simulink model "Homodyne_Tranceriver_model_v2"  (R2026b)
settings: Solver=VariableStepAuto  StopTime=16
libraries: fl_lib x10, nesl_utility x5, simrfV2util1 x4, simrfV2elements x4, simrfV2_lib x2, ee_lib x2, dspsigops x1, simulink_extras x1, simulink x1
settings Model: Creator=dylan  LastModifiedBy=dylan
settings SimscapeCC: SimscapeLogType=all  SimscapeNominalValues="[{\"value\":\"1\",\"unit\":\"A\"},{\"value\":\"1\",\"unit\":\"bar\"},{\"value\":\"1\",\"unit\":\"cm^2\"},{\"value\":\"1\",\"unit\":\"cm^3/s\"},{\"value\":\"1\",\"unit\":\"kJ/kg\"},{\"value\":\"1\",\"unit\":\"kW\"},{\"value\":\"1\",\"unit\":\"l\"},{\"value\":\"1\",\"unit\":\"N\"},{\"value\":\"1\",\"unit\":\"N*m\"},{\"value\":\"1\",\"unit\":\"V\"},{\"value\":\"0.001\",\"unit\":\"Wb\"}]"  SimscapeUseEnergyAccounting=off

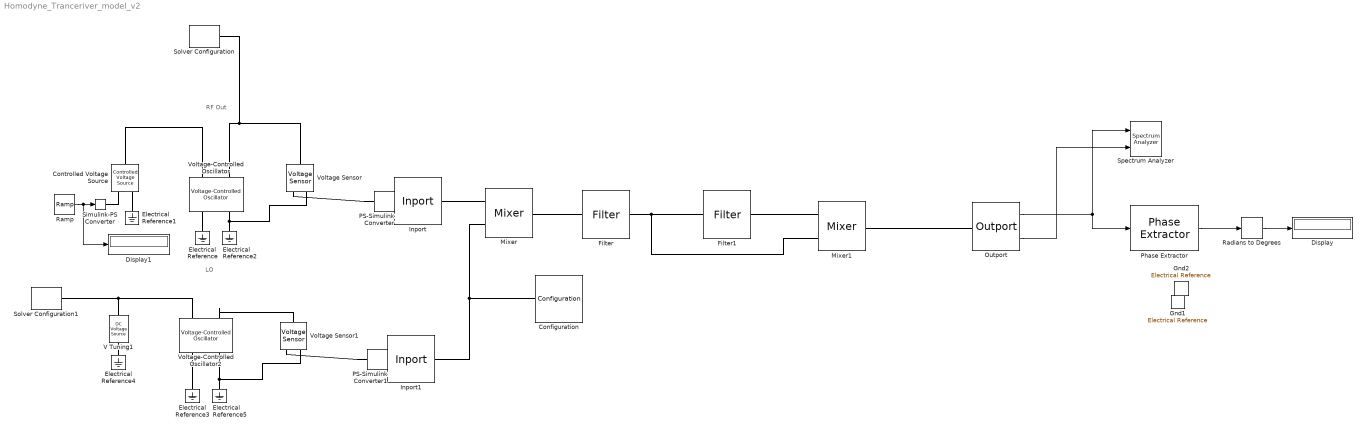
== system Homodyne_Tranceriver_model_v2 ==
  note: RF Out
  note: LO
  Configuration : simrfV2util1/Configuration  AutoFreq=on  Tones=[0] Hz  Harmonics=[1]  NormalizeCarrierPower=on  SolverType=Auto  UseCCode=on  StepSize=1 ns  AddNoise=on  defaultRNG=on  Seed=0  Temperature=290.0 K  SolverDelFlag=0  AbsTol=1e-6  RelTol=1e-3  MaxIter=10  ErrorEstimationType=2-norm over all variables  EnableInterpFilter=on  HiddenFIRfilterControllerParam=off  SmallSignalApprox=off  AllSimFreqs=on  SimFreqs=[] Hz  SimFreqsInternal=[]  SamplesPerFrame=1
  Controlled Voltage Source : fl_lib/Electrical/Electrical Sources/Controlled Voltage Source
  Display : Display
  Display1 : Display
  Electrical Reference{,1..5} (6 alike) : fl_lib/Electrical/Electrical Elements/Electrical Reference
  Filter : simrfV2elements/Filter  classname=filter  DesignMethod=Butterworth  ResponseType=Lowpass  Implementation=LC Tee  ImplementationIdeal=Constant per carrier  ImplementationRational=Transfer function  UseFilterOrder=on  FilterOrder=3  PassFreq_lp=150 MHz  PassFreq_hp=2 GHz  PassFreq_bp=[2 3] GHz  PassFreq_bs=[1 4] GHz  PassAtten=10*log10(2)  StopFreq_lp=2 GHz  StopFreq_hp=1 GHz  StopFreq_bp=[1.5 3.5] GHz  StopFreq_bs=[2.1 2.9] GHz  StopAtten=40  Rsrc=50  Rload=50  AutoImpulseLength=on  ImpulseLength=1e-10 s  InternalGrounding=on  PlotFuncLeft=Voltage transfer  PlotLeftForm=Magnitude (dB)  PlotRightOnVT=None  PlotRightNoTD=None  PlotRightNoGD=None  PlotRightNoIR=None  PlotRightNoSR=None  PlotRightForm=Magnitude (dB)  FreqPoints=logspace(0,10,101)  Freq_unit=Hz  TimePoints=linspace(0,1,1e6+1)  Time_unit=s  XaxisScale=Linear  YaxisScale=Linear  needRedraw=0
  Filter1 : simrfV2elements/Filter  classname=filter  DesignMethod=Ideal  ResponseType=Lowpass  Implementation=Transfer function  ImplementationIdeal=Frequency domain  ImplementationRational=Transfer function  UseFilterOrder=off  FilterOrder=3  PassFreq_lp=23.1 MHz  PassFreq_hp=2 GHz  PassFreq_bp=[2 3] GHz  PassFreq_bs=[1 4] GHz  PassAtten=10*log10(2)  StopFreq_lp=230 MHz  StopFreq_hp=1 GHz  StopFreq_bp=[1.5 3.5] GHz  StopFreq_bs=[2.1 2.9] GHz  StopAtten=20  Rsrc=50  Rload=50  AutoImpulseLength=on  ImpulseLength=1e-10 s  InternalGrounding=on  PlotFuncLeft=Voltage transfer  PlotLeftForm=Magnitude (dB)  PlotRightOnVT=None  PlotRightNoTD=None  PlotRightNoGD=None  PlotRightNoIR=None  PlotRightNoSR=None  PlotRightForm=Magnitude (dB)  FreqPoints=logspace(0,10,101)  Freq_unit=Hz  TimePoints=linspace(0,1,1e6+1)  Time_unit=s  XaxisScale=Linear  YaxisScale=Linear  needRedraw=1
  Gnd1 : simrfV2_lib/Elements/Electrical Reference
      settings: LibrarySourceBlock=simrfV2elements/Gnd
  Gnd2 : simrfV2_lib/Elements/Electrical Reference
      settings: LibrarySourceBlock=simrfV2elements/Gnd
  Inport : simrfV2util1/Inport  SimulinkInputSignalType=Ideal voltage  CarrierFreq=0 Hz  ZS=0  UseSqWave=off  NumCoeff=10  Bias=0  DutyCyc=50  AddNoise=off  InternalGrounding=on
  Inport1 : simrfV2util1/Inport  SimulinkInputSignalType=Ideal voltage  CarrierFreq=0 Hz  ZS=0  UseSqWave=off  NumCoeff=10  Bias=0  DutyCyc=50  AddNoise=off  InternalGrounding=on
  Mixer : simrfV2elements/Mixer  classname=mixer  Source_linear_gain=Available power gain  linear_gain=0 dB  Zin=50  Zout=50  ZLO=inf  Poly_Coeffs=[0 1]  IPType=Output  IP2=Inf dBm  IP3=Inf dBm  P1dB=Inf dBm  Psat=Inf dBm  Gcomp=Inf dBm  NF=0  InternalGrounding=on
  Mixer1 : simrfV2elements/Mixer  classname=mixer  Source_linear_gain=Available power gain  linear_gain=0 dB  Zin=50  Zout=50  ZLO=inf  Poly_Coeffs=[0 1]  IPType=Output  IP2=Inf dBm  IP3=Inf dBm  P1dB=Inf dBm  Psat=Inf dBm  Gcomp=Inf dBm  NF=0  InternalGrounding=on
  Outport : simrfV2util1/Outport  SensorType=Power  OutputFormat=Magnitude and Angle Baseband  CarrierFreq=0 Hz  ZL=50  AddNoise=off  InternalGrounding=on  StepSize=1e-09 s  AutoStep=on  HalfPolyphaseLength=12
  PS-Simulink Converter : nesl_utility/PS-Simulink Converter  PhysicalDomain=network_engine_domain  SubClassName=ps_output  LeftPortType=input  RightPortType=output  PseudoPeriodic=off  Frequencies=[]  VectorFormat=inherit  Unit=inherit  AffineConversion=off
  PS-Simulink Converter1 : nesl_utility/PS-Simulink Converter  PhysicalDomain=network_engine_domain  SubClassName=ps_output  LeftPortType=input  RightPortType=output  PseudoPeriodic=off  Frequencies=[]  VectorFormat=inherit  Unit=inherit  AffineConversion=off
  Phase Extractor : dspsigops/Phase Extractor  TreatFramesIndependently=on  SimulateUsing=Interpreted execution
  Radians to Degrees : simulink_extras/Transformations/Radians to Degrees
  Ramp : simulink/Sources/Ramp  slope=1  start=0  InitialOutput=1
  Simulink-PS Converter : nesl_utility/Simulink-PS Converter  PhysicalDomain=network_engine_domain  SubClassName=ps_input  LeftPortType=input  RightPortType=output  PseudoPeriodic=off  Frequencies=[]  NoiseDistribution=none  NoiseParameters=[]  Unit=1  AffineConversion=off  FilteringAndDerivatives=provide  SimscapeFilterOrder=1  InputFilterTimeConstant=0.001  UdotUserProvided=0
  Solver Configuration : nesl_utility/Solver Configuration  PhysicalDomain=network_engine_domain  SubClassName=solver  LeftPortType=input  RightPortType=generic  Tones=[]  Harmonics=[]  SimulateNoise=off  Profile=off  UseLocalSampling=off  EnableSwitchedLinearOptims=on  FrequencyDomain=off  UseCCode=off  RelTol=0.001  AbsTol=0.001  MinStep=1e-09  ToWorkspace=off  RevertToSquareIcSolve=off  NumHomotopyIterations=100  PhasorMode=off  PhasorModeNumHarmonics=1  ConsistencySolver=NEWTON_XTOL_AFTER_FTOL  CanonicalOrdering=CANONICAL  OptimizeIntermediates=OPTIMIZED  MulticoreSolverChoice=BACKWARD_EULER  IndexReductionMethod=DerivativeReplacement  DoDC=off  ResidualTolerance=1e-09  ConsistencyTolSource=GLOBAL  ConsistencyAbsTol=0.001  ConsistencyRelTol=0.001  ConsistencyTolFactor=0.001  UseLocalSolver=off  LocalSolverChoice=NE_BACKWARD_EULER_ADVANCER  ResolveIndetEquations=on  FunctionEvalNumThread=1  LocalSolverSampleTime=0.001  DoFixedCost=off  MaxNonlinIter=3  MaxModeIter=2  ComputeImpulses=off  ImpulseIterations=2  LinearAlgebra=auto  LinearAlgebraNumThread=0  EquationFormulation=NE_TIME_EF  DelaysMemoryBudget=1024  AutomaticFiltering=on  FilteringTimeConstant=0.001  PartitionStorageMethod=AS_NEEDED  PartitionMemoryBudget=1024  PartitionMethod=BALANCED  MultibodyUseLocalSolver=off  MultibodyLocalSolverChoice=ODE1  MultibodyLocalSolverSampleTime=0.001
  Solver Configuration1 : nesl_utility/Solver Configuration  PhysicalDomain=network_engine_domain  SubClassName=solver  LeftPortType=input  RightPortType=generic  Tones=[]  Harmonics=[]  SimulateNoise=off  Profile=off  UseLocalSampling=off  EnableSwitchedLinearOptims=on  FrequencyDomain=off  UseCCode=off  RelTol=0.001  AbsTol=0.001  MinStep=1e-09  ToWorkspace=off  RevertToSquareIcSolve=off  NumHomotopyIterations=100  PhasorMode=off  PhasorModeNumHarmonics=1  ConsistencySolver=NEWTON_XTOL_AFTER_FTOL  CanonicalOrdering=CANONICAL  OptimizeIntermediates=OPTIMIZED  MulticoreSolverChoice=BACKWARD_EULER  IndexReductionMethod=DerivativeReplacement  DoDC=off  ResidualTolerance=1e-09  ConsistencyTolSource=GLOBAL  ConsistencyAbsTol=0.001  ConsistencyRelTol=0.001  ConsistencyTolFactor=0.001  UseLocalSolver=off  LocalSolverChoice=NE_BACKWARD_EULER_ADVANCER  ResolveIndetEquations=on  FunctionEvalNumThread=1  LocalSolverSampleTime=0.001  DoFixedCost=off  MaxNonlinIter=3  MaxModeIter=2  ComputeImpulses=off  ImpulseIterations=2  LinearAlgebra=auto  LinearAlgebraNumThread=0  EquationFormulation=NE_TIME_EF  DelaysMemoryBudget=1024  AutomaticFiltering=on  FilteringTimeConstant=0.001  PartitionStorageMethod=AS_NEEDED  PartitionMemoryBudget=1024  PartitionMethod=BALANCED  MultibodyUseLocalSolver=off  MultibodyLocalSolverChoice=ODE1  MultibodyLocalSolverSampleTime=0.001
  Spectrum Analyzer : SpectrumAnalyzer  NumInputPorts=2  WindowPosition=[152.000000,116.000000,800.000000,500.000000,]  ScopeFrameLocation=window  SpectrumType=RMS  WindowInvariantSamplesPerUpdate=on  SpectrumUnits=Vrms  YLimits=[-1.601662291684014 2.886072017722371]  SelectedToolstripTab=spectrumAnalyzerToolstrip.homeTab
  V Tuning1 : fl_lib/Electrical/Electrical Sources/DC Voltage Source  v0=1 V
  Voltage Sensor : fl_lib/Electrical/Electrical Sensors/Voltage Sensor
  Voltage Sensor1 : fl_lib/Electrical/Electrical Sensors/Voltage Sensor
  Voltage-Controlled Oscillator : ee_lib/Integrated Circuits/Voltage-Controlled Oscillator  tabulated=ee.enum.ic.vcoFrequencyDependence.linear  f_nom=75 MHz  v_nom=1 V  df_dv=58000000 Hz/V  v_min=1 V  v_max=16 V  v_vec=[0, .2, .4, .6, .8, 1] V  f_vec=[-1000, -329, -51, 162, 342, 500] Hz  v_out=1 V  r_in=inf Ohm  r_out=50 Ohm  model_dynamics=ee.enum.ic.vcoDynamics.no  time_constant=1e-3 s  f_ini=1000 Hz
  Voltage-Controlled Oscillator2 : ee_lib/Integrated Circuits/Voltage-Controlled Oscillator  tabulated=ee.enum.ic.vcoFrequencyDependence.linear  f_nom=100 MHz  v_nom=1 V  df_dv=7700000 Hz/V  v_min=1 V  v_max=16 V  v_vec=[0, .2, .4, .6, .8, 1] V  f_vec=[-1000, -329, -51, 162, 342, 500] Hz  v_out=0.2 V  r_in=inf Ohm  r_out=50 Ohm  model_dynamics=ee.enum.ic.vcoDynamics.no  time_constant=1e-3 s  f_ini=1000 Hz
  wires:
  PS-Simulink Converter/1 -> Inport/1
  PS-Simulink Converter1/1 -> Inport1/1
  Outport/1 -> Phase Extractor/1, Spectrum Analyzer/1
  Ramp/1 -> Display1/1, Simulink-PS Converter/1
  Phase Extractor/1 -> Radians to Degrees/1
  Radians to Degrees/1 -> Display/1
  Outport/2 -> Spectrum Analyzer/2
  connections:
  Controlled Voltage Source/LConn1 -- Voltage-Controlled Oscillator/LConn1
  Electrical Reference/LConn1 -- Voltage-Controlled Oscillator/RConn1
  Controlled Voltage Source/RConn2 -- Electrical Reference1/LConn1
  Electrical Reference2/LConn1 -- Voltage Sensor/RConn2 -- Voltage-Controlled Oscillator/RConn2
  Voltage Sensor/LConn1 -- Solver Configuration/RConn1 -- Voltage-Controlled Oscillator/LConn2
  PS-Simulink Converter/LConn1 -- Voltage Sensor/RConn1
  Mixer/LConn1 -- Inport/RConn1
  Electrical Reference5/LConn1 -- Voltage Sensor1/RConn2 -- Voltage-Controlled Oscillator2/RConn2
  Electrical Reference4/LConn1 -- V Tuning1/RConn1
  PS-Simulink Converter1/LConn1 -- Voltage Sensor1/RConn1
  V Tuning1/LConn1 -- Voltage-Controlled Oscillator2/LConn1 -- Solver Configuration1/RConn1
  Electrical Reference3/LConn1 -- Voltage-Controlled Oscillator2/RConn1
  Inport1/RConn1 -- Mixer/LConn2 -- Configuration/LConn1
  Voltage-Controlled Oscillator2/LConn2 -- Voltage Sensor1/LConn1
  Filter/LConn1 -- Mixer/RConn1
  Filter/RConn1 -- Filter1/LConn1 -- Mixer1/LConn2
  Outport/LConn1 -- Mixer1/RConn1
  Simulink-PS Converter/RConn1 -- Controlled Voltage Source/RConn1
  Filter1/RConn1 -- Mixer1/LConn1
